simulink model "MMC_phase_centralized_HAAS_20260927"  (R2024b)
settings: Solver=FixedStepDiscrete  StartTime=t_init_sim  StopTime=sim_time  FixedStep=Ts  RelTol=1e-3
values from neighbouring files (symbols this model uses):
  a = 1    [script_MMC_phase_hackathon_NLM_centralized_HAAS_20260927.m]
  C1low1_active = 1    [script_MMC_phase_hackathon_NLM_centralized_HAAS_20260927.m]
  C2low1_active = 1    [script_MMC_phase_hackathon_NLM_centralized_HAAS_20260927.m]
  C_bus = 4400e-6    (= 0.0044)    [script_MMC_phase_hackathon_NLM_centralized_HAAS_20260927.m]
  C_M_extra = C_m-twist_high_side_C    [script_MMC_phase_hackathon_NLM_centralized_HAAS_20260927.m]
  duty_cycle = 1.0    (= 1)    [script_MMC_phase_hackathon_NLM_centralized_HAAS_20260927.m]
  f0 = 50    [script_MMC_phase_hackathon_NLM_centralized_HAAS_20260927.m]
  feeder_current_lower_rate_limit = -10    [script_MMC_phase_hackathon_NLM_centralized_HAAS_20260927.m]    (also in twist_parameters.m = -500)
  feeder_current_tab = [0.328 0.217 0.162 0.132 0.109 0.094 0.083 0.075 0.068 0.062 0.058 0.054 ... (42 elements, 14x3)]    [feeder_current.mat]
  feeder_current_upper_rate_limit = 0.386/(20e-3)    (= 19.3)    [twist_parameters.m]
  is6VExternallySupplied = true    [script_MMC_phase_hackathon_NLM_centralized_HAAS_20260927.m]
  isFeederJumperOpen = true    [script_MMC_phase_hackathon_NLM_centralized_HAAS_20260927.m]
  L_arm = 30e-3    (= 0.03)    [script_MMC_phase_hackathon_NLM_centralized_HAAS_20260927.m]
  m = 1    [script_MMC_phase_hackathon_NLM_centralized_HAAS_20260927.m]
  N = 5    [script_MMC_phase_hackathon_NLM_centralized_HAAS_20260927.m]
  power_losses = false    [script_MMC_phase_hackathon_NLM_centralized_HAAS_20260927.m]
  R = 15    [script_MMC_phase_hackathon_NLM_centralized_HAAS_20260927.m]
  R_arm = 0.2    [script_MMC_phase_hackathon_NLM_centralized_HAAS_20260927.m]
  source_V = 0    [script_MMC_phase_hackathon_NLM_centralized_HAAS_20260927.m]
  Tcom_sample = round(Tcom / Ts)    [script_MMC_phase_hackathon_NLM_centralized_HAAS_20260927.m]
  time_charge = 0.1    [script_MMC_phase_hackathon_NLM_centralized_HAAS_20260927.m]
  time_decharge = 1.5    [script_MMC_phase_hackathon_NLM_centralized_HAAS_20260927.m]
  Ts = 1e-6    (= 1e-06)    [script_MMC_phase_hackathon_NLM_centralized_HAAS_20260927.m]
  twist_data_acquisition_delay = 50e-9    (= 5e-08)    [script_MMC_phase_hackathon_NLM_centralized_HAAS_20260927.m]    (also in twist_parameters.m)
  twist_data_sampling_period = 1/twist_freq_data_sampling    (= 5e-05)    [script_MMC_phase_hackathon_NLM_centralized_HAAS_20260927.m]    (also in twist_parameters.m)
  twist_dead_time = 200e-9    (= 2e-07)    [twist_parameters.m]
  twist_freq_switching = 200e3    (= 200000)    [twist_parameters.m]
  twist_high_side_adc_R = 1/(1/2e6 + 1/2e6 + 1/(330e3+5.6e3))    (= 251272.836178)    [twist_parameters.m]
  twist_high_side_C = 33e-6*4 + 4.7e-6*12    (= 0.0001884)    [twist_parameters.m]
  twist_high_side_feeder_R = 47e3+4.7e3    (= 51700)    [twist_parameters.m]
  twist_high_side_rC = 0.1    [twist_parameters.m]
  twist_low_side_adc_R = 150e3+470    (= 150470)    [twist_parameters.m]
  twist_low_side_C_ceramic = 3*4.7e-6    (= 1.41e-05)    [twist_parameters.m]
  twist_low_side_C_electrolytic = 47e-6    (= 4.7e-05)    [twist_parameters.m]
  twist_low_side_L = 33e-6    (= 3.3e-05)    [twist_parameters.m]
  twist_low_side_rC = 700e-3    (= 0.7)    [twist_parameters.m]
  twist_low_side_rL = 20e-3    (= 0.02)    [twist_parameters.m]
  twist_R_VCC = (tau_VCC/twist_high_side_C  - twist_high_side_rC)/(1-(tau_VCC/twist_high_side_C - twist_high_side_rC)/R_parallel)    (= 1110.74997822)    [twist_parameters.m]
  VDC = 48    [script_MMC_phase_hackathon_NLM_centralized_HAAS_20260927.m]
undefined symbols (not defined in the file or in its folder): C_SM, feeder_current, gcbh, sps_rtmsupport, twist_low_side_lC
libraries: spsSeriesRLCBranchLib x135, spsTriangleGeneratorLib x60, spsMosfetLib x60, spsCurrentMeasurementLib x43, spsVoltageMeasurementLib x35, spsControlledCurrentSourceLib x30, spsDiodeLib x22, spsIdealSwitchLib x20, spsControlledVoltageSourceLib x1, spsGroundLib x1, spspowerguiLib x1
(part 1 of 22)
settings Model: Creator=ana  LastModifiedBy=ana

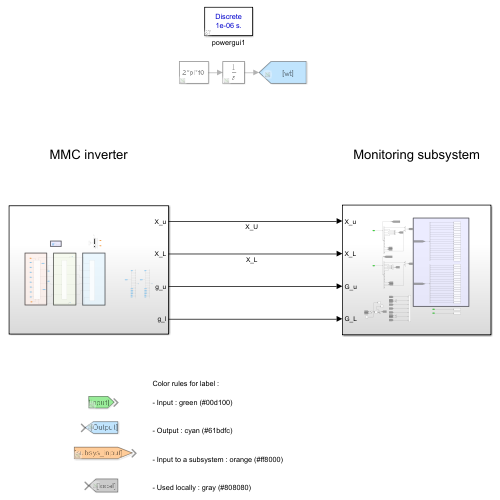
[thumbnail: Simulink's stored preview of the top-level diagram]
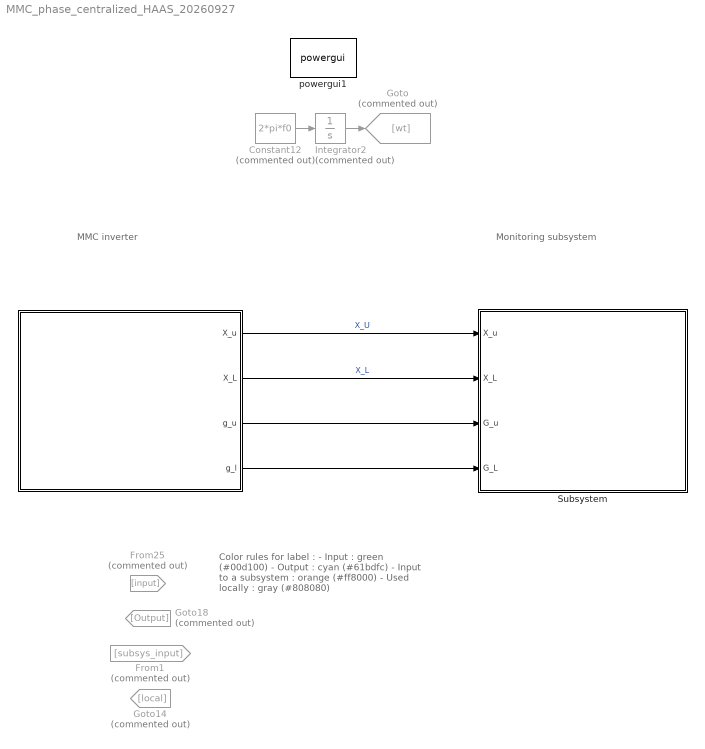
== system MMC_phase_centralized_HAAS_20260927 ==
  note: Color rules for label :
      |
      | - Input : green (#00d100)
      |
      |
      | - Output : cyan (#61bdfc)
      |
      |
      | - Input to a subsystem : orange (#ff8000)
      |
      |
      | - Used locally : gray (#808080)
  note: MMC inverter
  note: Monitoring subsystem
  " " : Subsystem
  Constant12 : Constant  Commented=on  Value=2*pi*f0
  From1 : From  Commented=on  GotoTag=subsys_input
  From25 : From  Commented=on  GotoTag=input
  Goto : Goto  Commented=on  GotoTag=wt
  Goto14 : Goto  Commented=on  GotoTag=local
  Goto18 : Goto  Commented=on  GotoTag=Output
  Integrator2 : Integrator  Commented=on
  Subsystem : Subsystem
  powergui1 : spspowerguiLib/powergui  Priority=1  SimulationMode=Discrete  SampleTime=Ts  frequency=60  Iterations=50  frequencyindice=0  Pbase=100e6  ErrMax=1e-4  UnitsV=V  UnitsW=W  buscounter=0  FunctionMessages=off  echomessages=off  EnableUseOfTLC=off  CurrentSourceSwitches=off  DisableSnubberDevices=off  DisableRonSwitches=off  DisableVfSwitches=off  DisplayEquations=off  AutomaticDiscreteSolvers=off  SolverType=Backward Euler  Interpol=off  ExternalGateDelay=off  methode=off  Ts=0  x0status=blocks  SPID=off  SwTol=0  HookPort=off  NonlinearTolerance=1e-4  nMaxIteration=100  ContinueOnMaxIteration=off  RestoreLinks=warning  ResistiveCurrentMeasurement=off  Frange=[0:2:500]  Ylog=off  Xlog=on  ShowGrid=off  save=off  variable=ZData  structure=0  ZoomFFT=off  StartTime=0.0  cycles=1  DisplayStyle=1  fundamental=60  FreqAxis=off  MaxFrequency=1000  frequencyindicesteady=1  RmsSteady=1  display=off
  wires:
  Constant12/1 -> Integrator2/1
  Integrator2/1 -> Goto/1
  " "/1(X_u) -> Subsystem/1(X_u)  "X_U"
  " "/2(X_L) -> Subsystem/2(X_L)  "X_L"
  " "/3(g_u) -> Subsystem/3(G_u)
  " "/4(g_l) -> Subsystem/4(G_L)

== system MMC_phase_centralized_HAAS_20260927/  ==
  note: Hardware
  note: Communication
  note: Power calculation
  note: Control
  Communication_subsystem : Subsystem
  Constant1 : Constant  Value=[1 1 1 1 1 1 1 1 1 1]
  Constant4 : Constant
  Constant5 : Constant  Value=[0 0 0 0 0 0 0 0 0 0]
  Demux : Demux  Outputs=10
  Demux3 : Demux  Outputs=10
  Demux4 : Demux  Outputs=10
  Mux1 : Mux  Inputs=17
  Mux{14..23} (10 alike) : Mux  Inputs=2
  Mux3 : Mux  Inputs=5
  Mux4 : Mux  Inputs=5
  Mux6 : Mux  Inputs=17
  Product1 : Product
  Sinus Modulation + Sorting Algorithm : Subsystem
      settings: PortSchema="{\"entries\":[{\"content\":{\"sides\":[{\"content\":{\"connectorIds\":[\"Out1\",\"In1\",\"In2\",\"In3\",\"In4\",\"Out2\"]},\"type\":\"ConnectorPlacement.EquallySpacedRectSide\",\"uuid\":\"ad0c70b8-bd3d-4dd9-a5c4-c9fd50c7c997\"},{\"content\":{\"side\":\"RIGHT\"},\"type\":\"ConnectorPlacement.EquallySpacedRectSide\",\"uuid\":\"9cc59a2e-07a9-40e0-b04f-27b582e27098\"},{\"content\":{\"side\":\"TOP\"},\"type\":\"ConnectorPlacement.EquallySpacedRectSide\",\"uuid\":\"c85123d6-aff8-40c6-b6df-c7fa366f0af5\"}]},\"type\":\"ConnectorPlacement.EquallySpacedConnector\",\"uuid\":\"b1891b87-83b0-4249-9289-dc35b8395afb\"}],\"packageUris\":[\"http://schema.mathworks.com/mf0/Connector/R2020b\"],\"version\":\"1.0\"}"
  Step2 : Step  Time=time_charge  SampleTime=Ts
  Subsystem : Subsystem
      settings: PortSchema="{\"entries\":[{\"content\":{\"sides\":[{\"content\":{\"connectorIds\":[\"Out7\",\"Out8\",\"Out9\",\"Out10\",\"Out11\",\"Out12\",\"Out13\",\"Out14\"]},\"type\":\"ConnectorPlacement.EquallySpacedRectSide\",\"uuid\":\"46d0b6b2-241e-4eaa-b5f4-7cb03ad6e4f0\"},{\"content\":{\"connectorIds\":[\"Out1\",\"Out2\",\"Out3\",\"Out4\",\"Out5\",\"Out6\"],\"side\":\"RIGHT\"},\"type\":\"ConnectorPlacement.EquallySpacedRectSide\",\"uuid\":\"f0391c40-5bbd-42ea-8549-0acba96c1793\"},{\"content\":{\"connectorIds\":[\"In1\",\"In2\"],\"side\":\"TOP\"},\"type\":\"ConnectorPlacement.EquallySpacedRectSide\",\"uuid\":\"1ede63b4-6869-46b3-8b67-84e7db18bcff\"},{\"content\":{\"connectorIds\":[\"In3\",\"In4\"],\"side\":\"BOTTOM\"},\"type\":\"ConnectorPlacement.EquallySpacedRectSide\",\"uuid\":\"c0e3b199-6126-45b0-9783-8fc4162e2280\"}]},\"type\":\"ConnectorPlacement.EquallySpacedConnector\",\"uuid\":\"8bedc799-aa9e-49e4-9c41-8dbcca404e51\"}],\"packageUris\":[\"http://schema.mathworks.com/mf0/Connector/R2020b\"],\"version\":\"1.0\"}"
  Switch2 : Switch  Criteria=u2 > Threshold  SaturateOnIntegerOverflow=off  InputSameDT=off
  To Workspace2 : ToWorkspace  VariableName=Pout  SaveFormat=Structure With Time  SampleTime=-1
  X_u : Outport
  X_L : Outport  Port=2
  g_u : Outport  Port=3
  g_l : Outport  Port=4
  wires:
  Mux6/1 -> X_u/1
  Sinus Modulation + Sorting Algorithm/1(gU) -> Subsystem/2(gU), g_u/1  "gU"
  Communication_subsystem/2(I_U_RX) -> Sinus Modulation + Sorting Algorithm/2(I_U)  "Iu_M1"
  Product1/1 -> To Workspace2/1  "P_sa"
  [iu] -> Product1/2
  [iu] -> Mux6/1  "Iu"
  [Vd_u] -> Mux6/12  "Vd_u"
  [N_u] -> Mux6/13  "N_u"
  [Vm_u] -> Mux6/14  "Vm_u"
  [v_a] -> Mux6/15  "V_s_a"
  [iu_M1] -> Mux6/16  "Iu_M1"
  [Vm_u] -> Product1/1
  Communication_subsystem/3(Vc_L_RX) -> Sinus Modulation + Sorting Algorithm/3(Vc_L)  "Vc_L"
  Sinus Modulation + Sorting Algorithm/2(gL) -> g_l/1, Subsystem/4(gL)  "gL"
  [il] -> Mux1/1  "iL"
  Mux1/1 -> X_L/1
  [il_M1] -> Mux1/16  "iL_M1"
  [Vd_l] -> Mux1/12  "Vd_l"
  [Vm_l] -> Mux1/14  "Vm_l"
  [N_l] -> Mux1/13  "N_l"
  [i_a] -> Mux1/15  "I_a"
  Communication_subsystem/4(I_L_RX) -> Sinus Modulation + Sorting Algorithm/4(I_L)  "IL_M1"
  Communication_subsystem/1(Vc_U_RX) -> Sinus Modulation + Sorting Algorithm/1(Vc_U)  "Vc_U"
  [Uppper_measure] -> Demux/1
  Demux/1 -> Mux6/2  "Vc_U_1"
  Demux/2 -> Mux6/3  "Vc_U_2"
  Demux/3 -> Mux6/4  "Vc_U_3"
  Demux/4 -> Mux6/5  "Vc_U_4"
  Demux/5 -> Mux6/6  "Vc_U_5"
  Demux/6 -> Mux6/7  "Vm_U_1"
  Demux/7 -> Mux6/8  "Vm_U_2"
  Demux/8 -> Mux6/9  "Vm_U_3"
  Demux/9 -> Mux6/10  "Vm_U_4"
  Demux/10 -> Mux6/11  "Vm_U_5"
  [Lower_measure] -> Demux3/1
  Demux3/1 -> Mux1/2  "Vc_L_1"
  Demux3/2 -> Mux1/3  "Vc_L_2"
  Demux3/3 -> Mux1/4  "Vc_L_3"
  Demux3/4 -> Mux1/5  "Vc_L_4"
  Demux3/5 -> Mux1/6  "Vc_L_5"
  Demux3/6 -> Mux1/7  "Vm_L_1"
  Demux3/7 -> Mux1/8  "Vm_L_2"
  Demux3/8 -> Mux1/9  "Vm_L_3"
  Demux3/9 -> Mux1/10  "Vm_L_4"
  Demux3/10 -> Mux1/11  "Vm_L_5"
  [m_u] -> Mux6/17  "m_u"
  [m_l] -> Mux1/17  "m_L"
  Subsystem/2(i_mod_M1) -> [iu_M1], Communication_subsystem/1(I_U_TX)  "IU_M1"
  Subsystem/4(i_mod_M6) -> [il_M1], Communication_subsystem/3(I_L_TX)  "IL_M6"
  Subsystem/6(Vc_L) -> Communication_subsystem/4(Vc_L_TX)
  Subsystem/3(Vc_U) -> Communication_subsystem/2(Vc_U_TX)  "Vc_U"
  Subsystem/10(i_a) -> [i_a]
  Subsystem/14(iu) -> [iu]
  Subsystem/8(Vm_u) -> [Vm_u]
  Subsystem/7(Vd_u) -> [Vd_u]
  Subsystem/12(il) -> [il]
  Subsystem/9(v_a) -> [v_a]
  Subsystem/13(Vd_l) -> [Vd_l]
  Subsystem/11(Vm_l) -> [Vm_l]
  Subsystem/5(Lower_measure) -> [Lower_measure]
  Subsystem/1(Upper_measure) -> [Uppper_measure]
  [block_U] -> Subsystem/1(block_U)
  [block_L] -> Subsystem/3(block_L)
  Demux4/9 -> Mux22/1  "block_L4"
  Mux17/1 -> Mux3/4
  Mux22/1 -> Mux4/4
  Mux14/1 -> Mux3/1
  Demux4/1 -> Mux14/1  "block_U1"
  Constant5/1 -> Switch2/1
  Demux4/3 -> Mux16/1  "block_U3"
  Mux21/1 -> Mux4/3
  Switch2/1 -> Demux4/1
  Demux4/5 -> Mux18/1  "block_U5"
  Demux4/10 -> Mux23/1  "block_L5"
  Constant1/1 -> Switch2/3
  Demux4/7 -> Mux20/1  "block_L2"
  Mux19/1 -> Mux4/1
  Mux23/1 -> Mux4/5
  Demux4/2 -> Mux15/1  "block_U2"
  Constant4/1 -> Mux23/2, Mux22/2, Mux21/2, Mux20/2, Mux19/2, Mux18/2, Mux17/2, Mux16/2, Mux15/2, Mux14/2
  Demux4/6 -> Mux19/1  "block_L1"
  Demux4/8 -> Mux21/1  "block_L3"
  Mux16/1 -> Mux3/3
  Mux15/1 -> Mux3/2
  Mux20/1 -> Mux4/2
  Mux18/1 -> Mux3/5
  Demux4/4 -> Mux17/1  "block_U4"
  Step2/1 -> Switch2/2
  Mux3/1 -> [block_U]
  Mux4/1 -> [block_L]

== system MMC_phase_centralized_HAAS_20260927/Subsystem ==
  note: To workspace
  X_u : Inport
  X_L : Inport  Port=2
  G_u : Inport  Port=3
  G_L : Inport  Port=4
  Constant : Constant  Value=2
  Demux : Demux  Outputs=2
  Demux{1..4} (4 alike) : Demux  Outputs=17
  Divide : Product  Inputs=*/
  Mux : Mux  Inputs=5
  Mux{1..3,8} (4 alike) : Mux  Inputs=2
  Mux5 : Mux  Inputs=5
  Scope : Scope
  Scope1 : Scope
  Scope3 : Scope  NumInputPorts=7
  Sum : Sum  Inputs=|++
  To Workspace1 : ToWorkspace  VariableName=vm_1  SaveFormat=Structure With Time  SampleTime=-1
  To Workspace10 : ToWorkspace  VariableName=vc_1  SaveFormat=Structure With Time  SampleTime=-1
  To Workspace11 : ToWorkspace  VariableName=va  SaveFormat=Structure With Time  SampleTime=-1
  To Workspace12 : ToWorkspace  VariableName=m_u  SaveFormat=Structure With Time  SampleTime=-1
  To Workspace13 : ToWorkspace  VariableName=i_u_M1_meas  SaveFormat=Structure With Time  SampleTime=-1
  To Workspace14 : ToWorkspace  VariableName=vm_10  SaveFormat=Structure With Time  SampleTime=-1
  To Workspace15 : ToWorkspace  VariableName=vm_2  SaveFormat=Structure With Time  SampleTime=-1
  To Workspace16 : ToWorkspace  VariableName=vm_3  SaveFormat=Structure With Time  SampleTime=-1
  To Workspace17 : ToWorkspace  VariableName=vm_4  SaveFormat=Structure With Time  SampleTime=-1
  To Workspace18 : ToWorkspace  VariableName=vm_5  SaveFormat=Structure With Time  SampleTime=-1
  To Workspace19 : ToWorkspace  VariableName=vc_10  SaveFormat=Structure With Time  SampleTime=-1
  To Workspace2 : ToWorkspace  VariableName=vc_2  SaveFormat=Structure With Time  SampleTime=-1
  To Workspace20 : ToWorkspace  VariableName=ia  SaveFormat=Structure With Time  SampleTime=-1
  To Workspace21 : ToWorkspace  VariableName=m_l  SaveFormat=Structure With Time  SampleTime=-1
  To Workspace22 : ToWorkspace  VariableName=i_l_M1_meas  SaveFormat=Structure With Time  SampleTime=-1
  To Workspace23 : ToWorkspace  VariableName=vm_6  SaveFormat=Structure With Time  SampleTime=-1
  To Workspace24 : ToWorkspace  VariableName=vm_7  SaveFormat=Structure With Time  SampleTime=-1
  To Workspace25 : ToWorkspace  VariableName=vm_8  SaveFormat=Structure With Time  SampleTime=-1
  To Workspace26 : ToWorkspace  VariableName=vm_9  SaveFormat=Structure With Time  SampleTime=-1
  To Workspace27 : ToWorkspace  VariableName=vc_6  SaveFormat=Structure With Time  SampleTime=-1
  To Workspace28 : ToWorkspace  VariableName=vc_7  SaveFormat=Structure With Time  SampleTime=-1
  To Workspace29 : ToWorkspace  VariableName=vc_8  SaveFormat=Structure With Time  SampleTime=-1
  To Workspace3 : ToWorkspace  VariableName=vc_3  SaveFormat=Structure With Time  SampleTime=-1
  To Workspace30 : ToWorkspace  VariableName=vc_9  SaveFormat=Structure With Time  SampleTime=-1
  To Workspace31 : ToWorkspace  VariableName=vd_l  SaveFormat=Structure With Time  SampleTime=-1
  To Workspace32 : ToWorkspace  VariableName=N_l  SaveFormat=Structure With Time  SampleTime=-1
  To Workspace33 : ToWorkspace  VariableName=i_l  SaveFormat=Structure With Time  SampleTime=-1
  To Workspace34 : ToWorkspace  VariableName=vm_l  SaveFormat=Structure With Time  SampleTime=-1
  To Workspace35 : ToWorkspace  VariableName=g_u  SaveFormat=Structure With Time  SampleTime=-1
  To Workspace36 : ToWorkspace  VariableName=g_L  SaveFormat=Structure With Time  SampleTime=-1
  To Workspace4 : ToWorkspace  VariableName=vc_4  SaveFormat=Structure With Time  SampleTime=-1
  To Workspace5 : ToWorkspace  VariableName=vc_5  SaveFormat=Structure With Time  SampleTime=-1
  To Workspace6 : ToWorkspace  VariableName=vd_u  SaveFormat=Structure With Time  SampleTime=-1
  To Workspace7 : ToWorkspace  VariableName=N_u  SaveFormat=Structure With Time  SampleTime=-1
  To Workspace8 : ToWorkspace  VariableName=i_u  SaveFormat=Structure With Time  SampleTime=-1
  To Workspace9 : ToWorkspace  VariableName=vm_u  SaveFormat=Structure With Time  SampleTime=-1
  wires:
  Demux4/15 -> To Workspace20/1  "i_a"
  Demux1/4 -> To Workspace3/1  "Vc_3"
  Demux4/17 -> To Workspace21/1  "m_l"
  X_L/1 -> Demux3/1, [l_SW]
  Demux2/14 -> [v_m_u]  "Vm_u"
  Demux1/2 -> To Workspace10/1  "Vc_1"
  Demux1/14 -> To Workspace9/1  "Vm_u"
  Mux2/1 -> Scope3/2  "V_m_U/L"
  Demux4/3 -> To Workspace28/1  "Vc_2"
  Demux1/7 -> To Workspace1/1  "Vm_1"
  Demux4/1 -> To Workspace33/1  "i_l"
  Demux2/1 -> Mux3/1  "i_u"
  Demux2/4 -> Mux/3  "V_uc_3"
  [v_m_u] -> Mux2/1
  [i_a] -> Scope3/7  "I_a"
  X_u/1 -> Demux2/1, [u_SW]
  Demux2/15 -> [v_a]  "V_a"
  Demux3/6 -> Mux5/5  "Vc_l_5"
  Demux2/16 -> Mux3/2  "iu_M1_meas"
  [i_l] -> Sum/2
  Demux3/1 -> Mux8/1  "i_l"
  Demux4/7 -> To Workspace23/1  "Vm_1"
  Demux1/11 -> To Workspace18/1  "Vm_5"
  Demux3/16 -> Mux8/2  "il_M1_meas"
  Demux1/13 -> To Workspace7/1  "N_u"
  Demux4/9 -> To Workspace25/1  "Vm_3"
  Demux2/3 -> Mux/2  "Vc_u_2"
  [i_u] -> Mux1/1
  Demux4/11 -> To Workspace14/1  "Vm_5"
  Mux5/1 -> [v_c_l]
  Demux4/8 -> To Workspace24/1  "Vm_2"
  [l_SW] -> Demux4/1  "L_SW"
  Demux1/5 -> To Workspace4/1  "Vc_4"
  Mux8/1 -> [i_l]
  Mux3/1 -> [i_u]  "I_u"
  Demux3/3 -> Mux5/2  "Vc_l_2"
  Constant/1 -> Divide/2
  Demux3/5 -> Mux5/4  "Vc_l_4"
  Demux4/4 -> To Workspace29/1  "Vc_3"
  Sum/1 -> Scope1/1, Divide/1  "I_u + I_L"
  Demux3/15 -> [i_a]  "i_a"
  Divide/1 -> Scope/1, Demux/1  "(I_U + I_L)/2"
  Demux1/3 -> To Workspace2/1  "Vc_2"
  Demux3/2 -> Mux5/1  "Vc_l_1"
  Demux1/16 -> To Workspace13/1  "iu_M1_meas"
  Demux2/5 -> Mux/4  "Vc_u_4"
  [v_a] -> Scope3/3  "V_a"
  Demux4/16 -> To Workspace22/1  "il_M1_meas"
  Demux1/10 -> To Workspace17/1  "Vm_4"
  [i_l] -> Mux1/2
  [u_SW] -> Demux1/1  "u_SW"
  Demux1/17 -> To Workspace12/1  "m_u"
  Demux1/15 -> To Workspace11/1  "Va"
  Demux1/12 -> To Workspace6/1  "Vd_u"
  Demux2/2 -> Mux/1  "Vc_u_1"
  Demux4/13 -> To Workspace32/1  "N_l"
  Demux1/9 -> To Workspace16/1  "Vm_3"
  Demux4/6 -> To Workspace19/1  "Vc_5"
  Demux4/2 -> To Workspace27/1  "Vc_1"
  Demux4/14 -> To Workspace34/1  "Vm_l"
  Demux/1 -> [i_Sigma_a]
  [v_c_l] -> Scope3/5  "V_c_L"
  Demux2/6 -> Mux/5  "Vc_u_5"
  Demux1/8 -> To Workspace15/1  "Vm_2"
  [v_c_u] -> Scope3/1  "V_c_u"
  Demux1/6 -> To Workspace5/1  "Vc_5"
  Demux1/1 -> To Workspace8/1  "i_u"
  [v_m_l] -> Mux2/2
  [i_u] -> Sum/1
  [i_Sigma_a] -> Scope3/4  "i_Sigma"
  Demux4/12 -> To Workspace31/1  "Vd_l"
  Demux3/14 -> [v_m_l]  "Vm_l"
  Mux1/1 -> Scope3/6  "I_U/L"
  Demux3/4 -> Mux5/3  "Vc_l_3"
  Mux/1 -> [v_c_u]  "V_c_u"
  Demux4/10 -> To Workspace26/1  "Vm_4"
  Demux4/5 -> To Workspace30/1  "Vc_4"
  G_u/1 -> To Workspace35/1
  G_L/1 -> To Workspace36/1

== system MMC_phase_centralized_HAAS_20260927/ /Communication_subsystem ==
  I_U_TX : Inport
  Vc_U_TX : Inport  Port=2
  I_L_TX : Inport  Port=3
  Vc_L_TX : Inport  Port=4
  Communication architecture : Subsystem
      settings: PortSchema="{\"entries\":[{\"content\":{\"sides\":[{\"content\":{\"connectorIds\":[\"In1\",\"Out2\",\"In2\",\"Out3\",\"In3\",\"Out4\",\"In4\",\"Out5\",\"In5\",\"Out6\",\"In6\",\"Out7\",\"In7\",\"Out8\",\"In8\",\"Out9\",\"In9\",\"Out10\",\"In10\",\"Out11\"]},\"type\":\"ConnectorPlacement.EquallySpacedRectSide\",\"uuid\":\"574f1c32-5c90-4713-aad2-348eca17c1e3\"},{\"content\":{\"connectorIds\":[\"Out1\"],\"side\":\"RIGHT\"},\"type\":\"ConnectorPlacement.EquallySpacedRectSide\",\"uuid\":\"f8c779b5-ecb7-4a42-bc9c-e4bb2f97a0b3\"},{\"content\":{\"side\":\"TOP\"},\"type\":\"ConnectorPlacement.EquallySpacedRectSide\",\"uuid\":\"aac8d141-a504-4135-a079-04baa73dba14\"}]},\"type\":\"ConnectorPlacement.EquallySpacedConnector\",\"uuid\":\"cbc34fff-d47b-42f9-bfde-18f06952df39\"}],\"packageUris\":[\"http://schema.mathworks.com/mf0/Connector/R2020b\"],\"version\":\"1.0\"}"
  Demux2 : Demux  Outputs=12
  Lower_arm : Subsystem
      settings: PortSchema="{\"entries\":[{\"content\":{\"sides\":[{\"content\":{\"connectorIds\":[\"In1\",\"In2\"]},\"type\":\"ConnectorPlacement.EquallySpacedRectSide\",\"uuid\":\"bca47161-c2bf-4caa-811b-3e74c86277e3\"},{\"content\":{\"connectorIds\":[\"Out1\",\"In3\",\"Out2\",\"In4\",\"Out3\",\"In5\",\"Out4\",\"In6\",\"Out5\",\"In7\"],\"side\":\"RIGHT\"},\"type\":\"ConnectorPlacement.EquallySpacedRectSide\",\"uuid\":\"b2e32fb7-723a-4edb-b512-e2e9b6c6de33\"},{\"content\":{\"side\":\"TOP\"},\"type\":\"ConnectorPlacement.EquallySpacedRectSide\",\"uuid\":\"c04e7617-ef7b-4140-bc2d-a2cc51392c69\"}]},\"type\":\"ConnectorPlacement.EquallySpacedConnector\",\"uuid\":\"316a164c-4e23-40e3-8762-9cd74b77f738\"}],\"packageUris\":[\"http://schema.mathworks.com/mf0/Connector/R2020b\"],\"version\":\"1.0\"}"
  Mux : Mux  Inputs=2
  Mux1 : Mux  Inputs=2
  Scope : Scope
  Sync : DiscretePulseGenerator  Period=round((200e-6)/Ts)  PulseWidth=round(20e-6/Ts)  SampleTime=Ts
  Upper_arm : Subsystem
      settings: PortSchema="{\"entries\":[{\"content\":{\"sides\":[{\"content\":{\"connectorIds\":[\"In1\",\"In2\"]},\"type\":\"ConnectorPlacement.EquallySpacedRectSide\",\"uuid\":\"e2448297-5920-4ed4-b9a5-463387ed0389\"},{\"content\":{\"connectorIds\":[\"Out1\",\"In3\",\"Out2\",\"In4\",\"Out3\",\"In5\",\"Out4\",\"In6\",\"Out5\",\"In7\"],\"side\":\"RIGHT\"},\"type\":\"ConnectorPlacement.EquallySpacedRectSide\",\"uuid\":\"29ac6558-0bf6-4432-86a8-2cc792ef1820\"},{\"content\":{\"connectorIds\":[\"Out6\"],\"side\":\"TOP\"},\"type\":\"ConnectorPlacement.EquallySpacedRectSide\",\"uuid\":\"fe3a666d-35d9-4a5d-8998-edcd1cd24e1f\"}]},\"type\":\"ConnectorPlacement.EquallySpacedConnector\",\"uuid\":\"a9564cd0-ea30-4b39-994d-f524846fcfc7\"}],\"packageUris\":[\"http://schema.mathworks.com/mf0/Connector/R2020b\"],\"version\":\"1.0\"}"
  Vector Concatenate : Concatenate  NumInputs=5
  Vector Concatenate1 : Concatenate  NumInputs=5
  Vc_U_RX : Outport
  I_U_RX : Outport  Port=2
  Vc_L_RX : Outport  Port=3
  I_L_RX : Outport  Port=4
  wires:
  Vc_U_TX/1 -> Mux/1
  Mux/1 -> Upper_arm/1(upper_arm_info)
  Vc_L_TX/1 -> Mux1/1
  I_L_TX/1 -> Mux1/2
  Mux1/1 -> Lower_arm/2(lower_arm_info)
  Upper_arm/1(M1_TX_signal) -> Communication architecture/1(M1_TX_Signal)
  Upper_arm/2(M2_TX_signal) -> Communication architecture/2(M2_TX_Signal)
  Upper_arm/3(M3_TX_signal) -> Communication architecture/3(M3_TX_Signal)
  Upper_arm/4(M4_TX_signal) -> Communication architecture/4(M4_TX_Signal)
  Upper_arm/5(M5_TX_signal) -> Communication architecture/5(M5_TX_Signal)
  Lower_arm/1(M6_TX_signal) -> Communication architecture/6(M6_TX_Signal)
  Lower_arm/2(M7_TX_signal) -> Communication architecture/7(M7_TX_Signal)
  Lower_arm/3(M8_TX_signal) -> Communication architecture/8(M8_TX_Signal)
  Lower_arm/4(M9_TX_signal) -> Communication architecture/9(M9_TX_Signal)
  Lower_arm/5(M10_TX_signal) -> Communication architecture/10(M10_TX_Signal)
  I_U_TX/1 -> Mux/2
  Sync/1 -> Lower_arm/1(sync), Upper_arm/2(sync)
  Upper_arm/6(RX_Variables) -> [RX_variable]
  [RX_variable] -> Demux2/1
  Demux2/1 -> Scope/1, Vector Concatenate/1  "Vc_u_1"
  Demux2/2 -> Vector Concatenate/2  "Vc_u_2"
  Demux2/3 -> Vector Concatenate/3  "Vc_u_3"
  Demux2/4 -> Vector Concatenate/4  "Vc_u_4"
  Demux2/5 -> Vector Concatenate/5  "Vc_u_5"
  Vector Concatenate/1 -> Vc_U_RX/1
  Demux2/6 -> I_U_RX/1
  Demux2/11 -> Vector Concatenate1/5  "Vc_l_5"
  Demux2/9 -> Vector Concatenate1/3  "Vc_l_3"
  Demux2/8 -> Vector Concatenate1/2  "Vc_l_2"
  Demux2/10 -> Vector Concatenate1/4  "Vc_l_4"
  Demux2/7 -> Vector Concatenate1/1  "Vc_l_1"
  Vector Concatenate1/1 -> Vc_L_RX/1
  Demux2/12 -> I_L_RX/1
  Communication architecture/2(M1_RX_Signal) -> Upper_arm/3(M1_RX_signal)
  Communication architecture/3(M2_RX_Signal) -> Upper_arm/4(M2_RX_signal)
  Communication architecture/4(M3_RX_Signal) -> Upper_arm/5(M3_RX_signal)
  Communication architecture/5(M4_RX_Signal) -> Upper_arm/6(M4_RX_signal)
  Communication architecture/6(M5_RX_Signal) -> Upper_arm/7(M5_RX_signal)
  Communication architecture/7(M6_RX_Signal) -> Lower_arm/3(M6_RX_signal)
  Communication architecture/8(M7_RX_Signal) -> Lower_arm/4(M7_RX_signal)
  Communication architecture/9(M8_RX_Signal) -> Lower_arm/5(M8_RX_signal)
  Communication architecture/10(M9_RX_Signal) -> Lower_arm/6(M9_RX_signal)
  Communication architecture/11(M10_RX_Signal) -> Lower_arm/7(M10_RX_signal)

== system MMC_phase_centralized_HAAS_20260927/ /Sinus Modulation + Sorting Algorithm ==
  note: Sorting and CVB algorithm - Upper and Lower stacks
  note: Gate assignement - Modules MCUs
  Vc_U : Inport
  I_U : Inport  Port=2
  Vc_L : Inport  Port=3
  I_L : Inport  Port=4
  Constant10 : Constant
  Constant11 : Constant  Value=2
  Constant12 : Constant  Value=3
  Constant13 : Constant  Value=4
  Constant14 : Constant  Value=5
  Constant5 : Constant
  Constant6 : Constant  Value=2
  Constant7 : Constant  Value=3
  Constant8 : Constant  Value=4
  Constant9 : Constant  Value=5
  M1 MCU : Subsystem
  M2 MCU : Subsystem
  M3 MCU : Subsystem
  M4 MCU : Subsystem
  M5 MCU : Subsystem
  M5 MCU1 : Subsystem
  M5 MCU2 : Subsystem
  M5 MCU3 : Subsystem
  M5 MCU4 : Subsystem
  M5 MCU5 : Subsystem
  Mux : Mux  Inputs=5
  Mux1 : Mux  Inputs=5
  Supervisor MCU : Subsystem
  gU : Outport
  gL : Outport  Port=2
  tag scope: g_l_supervisor=global, g_u_supervisor=global
  wires:
  M1 MCU/1(g_unitaire_stack) -> Mux/1
  M2 MCU/1(g_unitaire_stack) -> Mux/2
  M3 MCU/1(g_unitaire_stack) -> Mux/3
  M4 MCU/1(g_unitaire_stack) -> Mux/4
  M5 MCU/1(g_unitaire_stack) -> Mux/5
  Constant5/1 -> M1 MCU/2(M_number)
  Constant6/1 -> M2 MCU/2(M_number)
  Constant7/1 -> M3 MCU/2(M_number)
  Constant8/1 -> M4 MCU/2(M_number)
  Constant9/1 -> M5 MCU/2(M_number)
  M5 MCU3/1(g_unitaire_stack) -> Mux1/3
  M5 MCU4/1(g_unitaire_stack) -> Mux1/4
  M5 MCU5/1(g_unitaire_stack) -> Mux1/5
  Constant10/1 -> M5 MCU1/2(M_number)
  Constant11/1 -> M5 MCU2/2(M_number)
  Constant12/1 -> M5 MCU3/2(M_number)
  Constant13/1 -> M5 MCU4/2(M_number)
  Constant14/1 -> M5 MCU5/2(M_number)
  I_U/1 -> Supervisor MCU/2(I_U)
  Vc_U/1 -> Supervisor MCU/1(Vc_U)
  Vc_L/1 -> Supervisor MCU/3(Vc_L)
  I_L/1 -> Supervisor MCU/4(I_L)
  M5 MCU1/1(g_unitaire_stack) -> Mux1/1
  M5 MCU2/1(g_unitaire_stack) -> Mux1/2
  Supervisor MCU/1(gU) -> [g_u_supervisor]
  Supervisor MCU/2(gL) -> [g_l_supervisor]
  [g_u_supervisor] -> M5 MCU/1(g_u), M4 MCU/1(g_u), M3 MCU/1(g_u), M2 MCU/1(g_u), M1 MCU/1(g_u)
  [g_l_supervisor] -> M5 MCU5/1(g_u), M5 MCU4/1(g_u), M5 MCU3/1(g_u), M5 MCU2/1(g_u), M5 MCU1/1(g_u)
  Mux1/1 -> gL/1
  Mux/1 -> gU/1

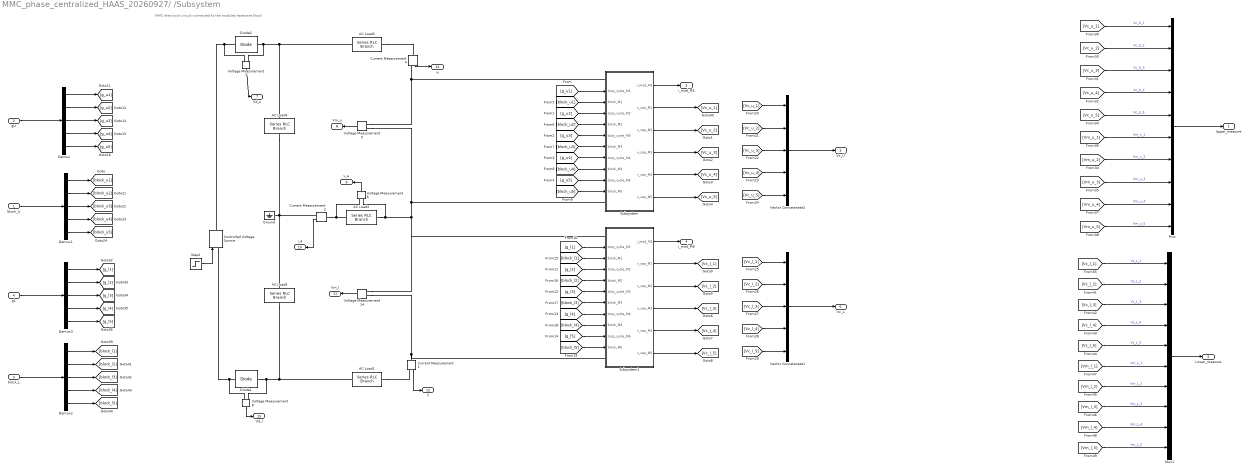
== system MMC_phase_centralized_HAAS_20260927/ /Subsystem ==
  note: MMC electrical circuit connected to the modules hardware block
  block_U : Inport
  gU : Inport  Port=2
  block_L : Inport  Port=3
  gL : Inport  Port=4
  AC Load1 : spsSeriesRLCBranchLib/Series RLC Branch  LConnTagsString=__new0  RConnTagsString=__new0  BranchType=RL  Resistance=R_arm  Inductance=L_arm  SetiL0=off  InitialCurrent=0  Capacitance=C_SM  Setx0=off  InitialVoltage=0  Measurements=None
  AC Load2 : spsSeriesRLCBranchLib/Series RLC Branch  LConnTagsString=__new0  RConnTagsString=__new0  BranchType=RL  Resistance=R_arm  Inductance=L_arm  SetiL0=off  InitialCurrent=0  Capacitance=C_SM  Setx0=off  InitialVoltage=0  Measurements=None
  AC Load3 : spsSeriesRLCBranchLib/Series RLC Branch  LConnTagsString=__new0  RConnTagsString=__new0  BranchType=R  Resistance=R  Inductance=L_arm  SetiL0=off  InitialCurrent=0  Capacitance=C_SM  Setx0=off  InitialVoltage=0  Measurements=None
  AC Load4 : spsSeriesRLCBranchLib/Series RLC Branch  LConnTagsString=__new0  RConnTagsString=__new0  BranchType=C  Resistance=R  Inductance=L_arm  SetiL0=off  InitialCurrent=0  Capacitance=C_bus  Setx0=off  InitialVoltage=0  Measurements=None
  AC Load5 : spsSeriesRLCBranchLib/Series RLC Branch  LConnTagsString=__new0  RConnTagsString=__new0  BranchType=C  Resistance=R  Inductance=L_arm  SetiL0=off  InitialCurrent=0  Capacitance=C_bus  Setx0=off  InitialVoltage=0  Measurements=None
  Controlled Voltage Source : spsControlledVoltageSourceLib/Controlled Voltage Source  Initialize=on  Source_Type=DC  Amplitude=0  Phase=0  Frequency=0  Measurements=None
  Current Measurement1 : spsCurrentMeasurementLib/Current Measurement  PhasorSimulation=off  OutputType=Complex  PSBequivalent=0
  Current Measurement2 : spsCurrentMeasurementLib/Current Measurement  PhasorSimulation=off  OutputType=Complex  PSBequivalent=0
  Current Measurement4 : spsCurrentMeasurementLib/Current Measurement  PhasorSimulation=off  OutputType=Complex  PSBequivalent=0
  Demux{,1..3} (4 alike) : Demux  Outputs=5
  Diode1 : spsDiodeLib/Diode  Ron=0.001  Lon=0  Vf=0.8  IC=0  UseSnubber=0  Rs=1e5  Cs=inf  Measurements=off
  Diode2 : spsDiodeLib/Diode  Ron=0.001  Lon=0  Vf=0.8  IC=0  UseSnubber=0  Rs=1e5  Cs=inf  Measurements=off
  Ground : spsGroundLib/Ground  LConnTagsString=a
  Mux : Mux  Inputs=10
  Mux1 : Mux  Inputs=10
  Step2 : Step  Time=time_decharge  Before=VDC  After=0  SampleTime=0
  Subsystem : Subsystem
      settings: PortSchema="{\"entries\":[{\"content\":{\"sides\":[{\"content\":{\"connectorIds\":[\"LConn1\",\"In1\",\"In2\",\"In3\",\"In4\",\"In5\",\"In6\",\"In7\",\"In8\",\"In9\",\"In10\",\"LConn2\"]},\"type\":\"ConnectorPlacement.EquallySpacedRectSide\",\"uuid\":\"af96ca56-9fdb-47ea-8e31-50f481daafc4\"},{\"content\":{\"connectorIds\":[\"Out1\",\"Out2\",\"Out3\",\"Out4\",\"Out5\",\"Out6\"],\"side\":\"RIGHT\"},\"type\":\"ConnectorPlacement.EquallySpacedRectSide\",\"uuid\":\"66f6256f-049a-4c8a-aad5-8d93b148b037\"},{\"content\":{\"side\":\"TOP\"},\"type\":\"ConnectorPlacement.EquallySpacedRectSide\",\"uuid\":\"596eb3e1-7761-4783-802e-d9df31b3a9c1\"}]},\"type\":\"ConnectorPlacement.EquallySpacedConnector\",\"uuid\":\"34c6ade5-a2f4-48d8-9a9b-6856a5a88d76\"}],\"packageUris\":[\"http://schema.mathworks.com/mf0/Connector/R2020b\"],\"version\":\"1.0\"}"
  Subsystem1 : Subsystem
      settings: PortSchema="{\"entries\":[{\"content\":{\"sides\":[{\"content\":{\"connectorIds\":[\"LConn1\",\"In1\",\"In2\",\"In3\",\"In4\",\"In5\",\"In6\",\"In7\",\"In8\",\"In9\",\"In10\",\"LConn2\"]},\"type\":\"ConnectorPlacement.EquallySpacedRectSide\",\"uuid\":\"af96ca56-9fdb-47ea-8e31-50f481daafc4\"},{\"content\":{\"connectorIds\":[\"Out1\",\"Out2\",\"Out3\",\"Out4\",\"Out5\",\"Out6\"],\"side\":\"RIGHT\"},\"type\":\"ConnectorPlacement.EquallySpacedRectSide\",\"uuid\":\"66f6256f-049a-4c8a-aad5-8d93b148b037\"},{\"content\":{\"side\":\"TOP\"},\"type\":\"ConnectorPlacement.EquallySpacedRectSide\",\"uuid\":\"596eb3e1-7761-4783-802e-d9df31b3a9c1\"}]},\"type\":\"ConnectorPlacement.EquallySpacedConnector\",\"uuid\":\"34c6ade5-a2f4-48d8-9a9b-6856a5a88d76\"}],\"packageUris\":[\"http://schema.mathworks.com/mf0/Connector/R2020b\"],\"version\":\"1.0\"}"
  Vector Concatenate1 : Concatenate  NumInputs=5
  Vector Concatenate2 : Concatenate  NumInputs=5
  Voltage Measurement{5..8,14} (5 alike) : spsVoltageMeasurementLib/Voltage Measurement  PhasorSimulation=off  OutputType=Complex  PSBequivalent=0
  Upper_measure : Outport
  i_mod_M1 : Outport  Port=2
  Vc_U : Outport  Port=3
  i_mod_M6 : Outport  Port=4
  Lower_measure : Outport  Port=5
  Vc_L : Outport  Port=6
  Vd_u : Outport  Port=7
  Vm_u : Outport  Port=8
  v_a : Outport  Port=9
  i_a : Outport  Port=10
  Vm_l : Outport  Port=11
  il : Outport  Port=12
  Vd_l : Outport  Port=13
  iu : Outport  Port=14
  wires:
  Voltage Measurement7/1 -> Vd_u/1
  Current Measurement2/1 -> i_a/1
  Step2/1 -> Controlled Voltage Source/1
  Voltage Measurement5/1 -> Vm_u/1
  Voltage Measurement6/1 -> v_a/1
  Voltage Measurement14/1 -> Vm_l/1
  [g_u1] -> Subsystem/1(duty_cycle_M1)
  [block_u1] -> Subsystem/2(block_M1)
  [g_u2] -> Subsystem/3(duty_cycle_M2)
  [block_u2] -> Subsystem/4(block_M2)
  [g_u3] -> Subsystem/5(duty_cycle_M3)
  [block_u3] -> Subsystem/6(block_M3)
  [g_u4] -> Subsystem/7(duty_cycle_M4)
  [block_u4] -> Subsystem/8(block_M4)
  [g_u5] -> Subsystem/9(duty_cycle_M5)
  [block_u5] -> Subsystem/10(block_M5)
  Subsystem/1(i_mod_M1) -> i_mod_M1/1
  Subsystem/6(v_cap_M5) -> [Vc_u_5]
  Subsystem/5(v_cap_M4) -> [Vc_u_4]
  Subsystem/2(v_cap_M1) -> [Vc_u_1]
  Subsystem/3(v_cap_M2) -> [Vc_u_2]
  Subsystem/4(v_cap_M3) -> [Vc_u_3]
  [block_l4] -> Subsystem1/8(block_M4)
  [g_l4] -> Subsystem1/7(duty_cycle_M4)
  [block_l5] -> Subsystem1/10(block_M5)
  [g_l5] -> Subsystem1/9(duty_cycle_M5)
  [g_l1] -> Subsystem1/1(duty_cycle_M1)
  [g_l2] -> Subsystem1/3(duty_cycle_M2)
  [block_l2] -> Subsystem1/4(block_M2)
  [g_l3] -> Subsystem1/5(duty_cycle_M3)
  [block_l1] -> Subsystem1/2(block_M1)
  [block_l3] -> Subsystem1/6(block_M3)
  Subsystem1/1(i_mod_M1) -> i_mod_M6/1
  Subsystem1/2(v_cap_M1) -> [Vc_l_1]
  Subsystem1/3(v_cap_M2) -> [Vc_l_2]
  Subsystem1/4(v_cap_M3) -> [Vc_l_3]
  Subsystem1/5(v_cap_M4) -> [Vc_l_4]
  Subsystem1/6(v_cap_M5) -> [Vc_l_5]
  Current Measurement4/1 -> iu/1
  Voltage Measurement8/1 -> Vd_l/1
  Current Measurement1/1 -> il/1
  Vector Concatenate2/1 -> Vc_U/1
  Demux/2 -> [g_u2]
  Demux/5 -> [g_u5]
  Demux1/5 -> [block_u5]
  Demux/4 -> [g_u4]
  Demux/3 -> [g_u3]
  Demux1/1 -> [block_u1]
  gU/1 -> Demux/1
  block_U/1 -> Demux1/1
  Demux1/2 -> [block_u2]
  Demux/1 -> [g_u1]
  Demux1/4 -> [block_u4]
  Demux1/3 -> [block_u3]
  Demux3/3 -> [g_l3]
  Demux3/4 -> [g_l4]
  Demux2/3 -> [block_l3]
  Demux2/1 -> [block_l1]
  Demux3/1 -> [g_l1]
  gL/1 -> Demux3/1
  Demux2/2 -> [block_l2]
  Demux2/4 -> [block_l4]
  Demux2/5 -> [block_l5]
  Demux3/5 -> [g_l5]
  block_L/1 -> Demux2/1
  Demux3/2 -> [g_l2]
  [Vc_u_1] -> Vector Concatenate2/1
  [Vc_u_2] -> Vector Concatenate2/2
  [Vc_u_3] -> Vector Concatenate2/3
  [Vc_u_4] -> Vector Concatenate2/4
  [Vc_u_5] -> Vector Concatenate2/5
  [Vc_l_5] -> Vector Concatenate1/5
  [Vc_l_1] -> Vector Concatenate1/1
  [Vc_l_4] -> Vector Concatenate1/4
  Vector Concatenate1/1 -> Vc_L/1
  [Vc_l_3] -> Vector Concatenate1/3
  [Vc_l_2] -> Vector Concatenate1/2
  [Vc_u_1] -> Mux/1  "Vc_U_1"
  [Vm_u_5] -> Mux/10  "Vm_u_5"
  [Vm_u_4] -> Mux/9  "Vm_u_4"
  [Vc_u_3] -> Mux/3  "Vc_U_3"
  [Vm_u_3] -> Mux/8  "Vm_u_3"
  [Vc_u_2] -> Mux/2  "Vc_U_2"
  [Vm_u_2] -> Mux/7  "Vm_u_2"
  [Vm_u_1] -> Mux/6  "Vm_u_1"
  [Vc_u_4] -> Mux/4  "Vc_U_4"
  [Vc_u_5] -> Mux/5  "Vc_U_5"
  [Vc_l_2] -> Mux1/2  "Vc_L_2"
  [Vm_l_2] -> Mux1/7  "Vm_L_2"
  [Vc_l_1] -> Mux1/1  "Vc_L_1"
  [Vm_l_4] -> Mux1/9  "Vm_L_4"
  [Vm_l_5] -> Mux1/10  "Vm_L_5"
  [Vm_l_1] -> Mux1/6  "Vm_L_1"
  [Vm_l_3] -> Mux1/8  "Vm_L_3"
  [Vc_l_3] -> Mux1/3  "Vc_L_3"
  [Vc_l_5] -> Mux1/5  "Vc_L_5"
  [Vc_l_4] -> Mux1/4  "Vc_L_4"
  Mux1/1 -> Lower_measure/1
  Mux/1 -> Upper_measure/1
  connections:
  Controlled Voltage Source/LConn1 -- Voltage Measurement8/LConn2 -- Diode1/RConn1
  AC Load2/LConn1 -- AC Load4/LConn1 -- Diode2/RConn1 -- Voltage Measurement7/LConn2
  Current Measurement4/RConn1 -- Voltage Measurement5/LConn1 -- Subsystem/LConn1
  Voltage Measurement14/LConn2 -- Subsystem1/LConn2 -- Current Measurement1/LConn1
  AC Load2/RConn1 -- Current Measurement4/LConn1
  Voltage Measurement6/LConn1 -- Subsystem1/LConn1 -- Voltage Measurement14/LConn1 -- Voltage Measurement5/LConn2 -- Subsystem/LConn2 -- AC Load3/RConn1
  Ground/LConn1 -- AC Load5/LConn1 -- AC Load4/RConn1 -- Current Measurement2/RConn1
  AC Load1/RConn1 -- Current Measurement1/RConn1
  Voltage Measurement7/LConn1 -- Controlled Voltage Source/RConn1 -- Diode2/LConn1
  AC Load1/LConn1 -- Diode1/LConn1 -- Voltage Measurement8/LConn1 -- AC Load5/RConn1
  Current Measurement2/LConn1 -- Voltage Measurement6/LConn2 -- AC Load3/LConn1

== system MMC_phase_centralized_HAAS_20260927/ /Communication_subsystem/Communication architecture ==
  M1_TX_Signal : Inport
  M2_TX_Signal : Inport  Port=2
  M3_TX_Signal : Inport  Port=3
  M4_TX_Signal : Inport  Port=4
  M5_TX_Signal : Inport  Port=5
  M6_TX_Signal : Inport  Port=6
  M7_TX_Signal : Inport  Port=7
  M8_TX_Signal : Inport  Port=8
  M9_TX_Signal : Inport  Port=9
  M10_TX_Signal : Inport  Port=10
  MATLAB Function : MATLAB Function  Commented=on  TreatAsAtomicUnit=on
  RX_Signal : Outport
  M1_RX_Signal : Outport  Port=2
  M2_RX_Signal : Outport  Port=3
  M3_RX_Signal : Outport  Port=4
  M4_RX_Signal : Outport  Port=5
  M5_RX_Signal : Outport  Port=6
  M6_RX_Signal : Outport  Port=7
  M7_RX_Signal : Outport  Port=8
  M8_RX_Signal : Outport  Port=9
  M9_RX_Signal : Outport  Port=10
  M10_RX_Signal : Outport  Port=11
  wires:
  MATLAB Function/1(bus_signal) -> RX_Signal/1
  M4_TX_Signal/1 -> M5_RX_Signal/1
  M5_TX_Signal/1 -> M6_RX_Signal/1
  M6_TX_Signal/1 -> M7_RX_Signal/1
  M7_TX_Signal/1 -> M8_RX_Signal/1
  M8_TX_Signal/1 -> M9_RX_Signal/1
  M9_TX_Signal/1 -> M10_RX_Signal/1
  M10_TX_Signal/1 -> M1_RX_Signal/1
  M1_TX_Signal/1 -> M2_RX_Signal/1
  M2_TX_Signal/1 -> M3_RX_Signal/1
  M3_TX_Signal/1 -> M4_RX_Signal/1

== system MMC_phase_centralized_HAAS_20260927/ /Communication_subsystem/Lower_arm ==
  sync : Inport
  lower_arm_info : Inport  Port=2
  M6_RX_signal : Inport  Port=3
  M7_RX_signal : Inport  Port=4
  M8_RX_signal : Inport  Port=5
  M9_RX_signal : Inport  Port=6
  M10_RX_signal : Inport  Port=7
  M1_Comm : Subsystem
      settings: PortSchema="{\"entries\":[{\"content\":{\"sides\":[{\"content\":{\"connectorIds\":[\"In1\",\"Out2\"]},\"type\":\"ConnectorPlacement.EquallySpacedRectSide\",\"uuid\":\"47077a1e-eba1-4129-8203-93262b2de465\"},{\"content\":{\"connectorIds\":[\"Out1\",\"In3\"],\"side\":\"RIGHT\"},\"type\":\"ConnectorPlacement.EquallySpacedRectSide\",\"uuid\":\"701fdbad-c928-45f3-8ba2-a14f680316f8\"},{\"content\":{\"side\":\"TOP\"},\"type\":\"ConnectorPlacement.EquallySpacedRectSide\",\"uuid\":\"d648951b-caea-4569-a411-8455254fdbc0\"},{\"content\":{\"connectorIds\":[\"In2\"],\"side\":\"BOTTOM\"},\"type\":\"ConnectorPlacement.EquallySpacedRectSide\",\"uuid\":\"07eb9aa1-f407-41f0-8942-d6ed405114b5\"}]},\"type\":\"ConnectorPlacement.EquallySpacedConnector\",\"uuid\":\"7c33ff72-602e-419f-9c2d-5eefc0d60400\"}],\"packageUris\":[\"http://schema.mathworks.com/mf0/Connector/R2020b\"],\"version\":\"1.0\"}"
  M2_Comm : Subsystem
      settings: PortSchema="{\"entries\":[{\"content\":{\"sides\":[{\"content\":{\"connectorIds\":[\"In1\",\"Out2\"]},\"type\":\"ConnectorPlacement.EquallySpacedRectSide\",\"uuid\":\"47077a1e-eba1-4129-8203-93262b2de465\"},{\"content\":{\"connectorIds\":[\"Out1\",\"In3\"],\"side\":\"RIGHT\"},\"type\":\"ConnectorPlacement.EquallySpacedRectSide\",\"uuid\":\"701fdbad-c928-45f3-8ba2-a14f680316f8\"},{\"content\":{\"side\":\"TOP\"},\"type\":\"ConnectorPlacement.EquallySpacedRectSide\",\"uuid\":\"d648951b-caea-4569-a411-8455254fdbc0\"},{\"content\":{\"connectorIds\":[\"In2\"],\"side\":\"BOTTOM\"},\"type\":\"ConnectorPlacement.EquallySpacedRectSide\",\"uuid\":\"01601a56-4c3c-4c18-be21-822f443ca232\"}]},\"type\":\"ConnectorPlacement.EquallySpacedConnector\",\"uuid\":\"7c33ff72-602e-419f-9c2d-5eefc0d60400\"}],\"packageUris\":[\"http://schema.mathworks.com/mf0/Connector/R2020b\"],\"version\":\"1.0\"}"
  M3_Comm : Subsystem
      settings: PortSchema="{\"entries\":[{\"content\":{\"sides\":[{\"content\":{\"connectorIds\":[\"In1\",\"Out2\"]},\"type\":\"ConnectorPlacement.EquallySpacedRectSide\",\"uuid\":\"47077a1e-eba1-4129-8203-93262b2de465\"},{\"content\":{\"connectorIds\":[\"Out1\",\"In3\"],\"side\":\"RIGHT\"},\"type\":\"ConnectorPlacement.EquallySpacedRectSide\",\"uuid\":\"701fdbad-c928-45f3-8ba2-a14f680316f8\"},{\"content\":{\"side\":\"TOP\"},\"type\":\"ConnectorPlacement.EquallySpacedRectSide\",\"uuid\":\"d648951b-caea-4569-a411-8455254fdbc0\"},{\"content\":{\"connectorIds\":[\"In2\"],\"side\":\"BOTTOM\"},\"type\":\"ConnectorPlacement.EquallySpacedRectSide\",\"uuid\":\"b7518228-bb66-4696-b5d4-126a1140e1c3\"}]},\"type\":\"ConnectorPlacement.EquallySpacedConnector\",\"uuid\":\"7c33ff72-602e-419f-9c2d-5eefc0d60400\"}],\"packageUris\":[\"http://schema.mathworks.com/mf0/Connector/R2020b\"],\"version\":\"1.0\"}"
  M4_Comm : Subsystem
      settings: PortSchema="{\"entries\":[{\"content\":{\"sides\":[{\"content\":{\"connectorIds\":[\"In1\",\"Out2\"]},\"type\":\"ConnectorPlacement.EquallySpacedRectSide\",\"uuid\":\"47077a1e-eba1-4129-8203-93262b2de465\"},{\"content\":{\"connectorIds\":[\"Out1\",\"In3\"],\"side\":\"RIGHT\"},\"type\":\"ConnectorPlacement.EquallySpacedRectSide\",\"uuid\":\"701fdbad-c928-45f3-8ba2-a14f680316f8\"},{\"content\":{\"side\":\"TOP\"},\"type\":\"ConnectorPlacement.EquallySpacedRectSide\",\"uuid\":\"d648951b-caea-4569-a411-8455254fdbc0\"},{\"content\":{\"connectorIds\":[\"In2\"],\"side\":\"BOTTOM\"},\"type\":\"ConnectorPlacement.EquallySpacedRectSide\",\"uuid\":\"5f4b38d1-ea61-4297-b8b6-4cb7ffcc6410\"}]},\"type\":\"ConnectorPlacement.EquallySpacedConnector\",\"uuid\":\"7c33ff72-602e-419f-9c2d-5eefc0d60400\"}],\"packageUris\":[\"http://schema.mathworks.com/mf0/Connector/R2020b\"],\"version\":\"1.0\"}"
  M5_Comm : Subsystem
      settings: PortSchema="{\"entries\":[{\"content\":{\"sides\":[{\"content\":{\"connectorIds\":[\"In1\",\"Out2\"]},\"type\":\"ConnectorPlacement.EquallySpacedRectSide\",\"uuid\":\"47077a1e-eba1-4129-8203-93262b2de465\"},{\"content\":{\"connectorIds\":[\"Out1\",\"In3\"],\"side\":\"RIGHT\"},\"type\":\"ConnectorPlacement.EquallySpacedRectSide\",\"uuid\":\"701fdbad-c928-45f3-8ba2-a14f680316f8\"},{\"content\":{\"side\":\"TOP\"},\"type\":\"ConnectorPlacement.EquallySpacedRectSide\",\"uuid\":\"d648951b-caea-4569-a411-8455254fdbc0\"},{\"content\":{\"connectorIds\":[\"In2\"],\"side\":\"BOTTOM\"},\"type\":\"ConnectorPlacement.EquallySpacedRectSide\",\"uuid\":\"cd08f752-2006-4da0-88d6-bb4b20ac3ab7\"}]},\"type\":\"ConnectorPlacement.EquallySpacedConnector\",\"uuid\":\"7c33ff72-602e-419f-9c2d-5eefc0d60400\"}],\"packageUris\":[\"http://schema.mathworks.com/mf0/Connector/R2020b\"],\"version\":\"1.0\"}"
  M6_TX_signal : Outport
  M7_TX_signal : Outport  Port=2
  M8_TX_signal : Outport  Port=3
  M9_TX_signal : Outport  Port=4
  M10_TX_signal : Outport  Port=5
  wires:
  [lower_arm_info] -> M5_Comm/1(TX_variables)
  M4_Comm/1(TX_signal) -> M9_TX_signal/1
  [lower_arm_info] -> M1_Comm/1(TX_variables)
  [lower_arm_info] -> M4_Comm/1(TX_variables)
  M3_Comm/1(TX_signal) -> M8_TX_signal/1
  M2_Comm/1(TX_signal) -> M7_TX_signal/1
  [lower_arm_info] -> M2_Comm/1(TX_variables)
  [lower_arm_info] -> M3_Comm/1(TX_variables)
  M6_RX_signal/1 -> M1_Comm/3(RX_signal)
  [sync] -> M3_Comm/2(sync)
  M8_RX_signal/1 -> M3_Comm/3(RX_signal)
  [sync] -> M5_Comm/2(sync)
  [sync] -> M4_Comm/2(sync)
  [sync] -> M1_Comm/2(sync)
  M10_RX_signal/1 -> M5_Comm/3(RX_signal)
  M1_Comm/1(TX_signal) -> M6_TX_signal/1
  M7_RX_signal/1 -> M2_Comm/3(RX_signal)
  [sync] -> M2_Comm/2(sync)
  M5_Comm/1(TX_signal) -> M10_TX_signal/1
  M9_RX_signal/1 -> M4_Comm/3(RX_signal)
  lower_arm_info/1 -> [lower_arm_info]
  sync/1 -> [sync]

== system MMC_phase_centralized_HAAS_20260927/ /Communication_subsystem/Upper_arm ==
  upper_arm_info : Inport
  sync : Inport  Port=2
  M1_RX_signal : Inport  Port=3
  M2_RX_signal : Inport  Port=4
  M3_RX_signal : Inport  Port=5
  M4_RX_signal : Inport  Port=6
  M5_RX_signal : Inport  Port=7
  M1_Comm : Subsystem
      settings: PortSchema="{\"entries\":[{\"content\":{\"sides\":[{\"content\":{\"connectorIds\":[\"In1\",\"Out2\"]},\"type\":\"ConnectorPlacement.EquallySpacedRectSide\",\"uuid\":\"c3733cfa-9814-4ae5-a55a-8e5b6f8a57d7\"},{\"content\":{\"connectorIds\":[\"Out1\",\"In3\"],\"side\":\"RIGHT\"},\"type\":\"ConnectorPlacement.EquallySpacedRectSide\",\"uuid\":\"d16535d3-81ee-4162-a646-15cef1f1639a\"},{\"content\":{\"side\":\"TOP\"},\"type\":\"ConnectorPlacement.EquallySpacedRectSide\",\"uuid\":\"672d53ef-99b6-4fa6-8351-42251f607454\"},{\"content\":{\"connectorIds\":[\"In2\"],\"side\":\"BOTTOM\"},\"type\":\"ConnectorPlacement.EquallySpacedRectSide\",\"uuid\":\"a9bd7512-44c2-4af9-8132-4c17be33b3c2\"}]},\"type\":\"ConnectorPlacement.EquallySpacedConnector\",\"uuid\":\"554aea8b-7fd0-4035-ac75-3acab423d605\"}],\"packageUris\":[\"http://schema.mathworks.com/mf0/Connector/R2020b\"],\"version\":\"1.0\"}"
  M2_Comm : Subsystem
      settings: PortSchema="{\"entries\":[{\"content\":{\"sides\":[{\"content\":{\"connectorIds\":[\"In1\",\"Out2\"]},\"type\":\"ConnectorPlacement.EquallySpacedRectSide\",\"uuid\":\"47077a1e-eba1-4129-8203-93262b2de465\"},{\"content\":{\"connectorIds\":[\"Out1\",\"In3\"],\"side\":\"RIGHT\"},\"type\":\"ConnectorPlacement.EquallySpacedRectSide\",\"uuid\":\"701fdbad-c928-45f3-8ba2-a14f680316f8\"},{\"content\":{\"side\":\"TOP\"},\"type\":\"ConnectorPlacement.EquallySpacedRectSide\",\"uuid\":\"d648951b-caea-4569-a411-8455254fdbc0\"},{\"content\":{\"connectorIds\":[\"In2\"],\"side\":\"BOTTOM\"},\"type\":\"ConnectorPlacement.EquallySpacedRectSide\",\"uuid\":\"d4b1d2d6-b4a1-4e2c-9ca6-248db102ef7c\"}]},\"type\":\"ConnectorPlacement.EquallySpacedConnector\",\"uuid\":\"7c33ff72-602e-419f-9c2d-5eefc0d60400\"}],\"packageUris\":[\"http://schema.mathworks.com/mf0/Connector/R2020b\"],\"version\":\"1.0\"}"
  M3_Comm : Subsystem
      settings: PortSchema="{\"entries\":[{\"content\":{\"sides\":[{\"content\":{\"connectorIds\":[\"In1\",\"Out2\"]},\"type\":\"ConnectorPlacement.EquallySpacedRectSide\",\"uuid\":\"47077a1e-eba1-4129-8203-93262b2de465\"},{\"content\":{\"connectorIds\":[\"Out1\",\"In3\"],\"side\":\"RIGHT\"},\"type\":\"ConnectorPlacement.EquallySpacedRectSide\",\"uuid\":\"701fdbad-c928-45f3-8ba2-a14f680316f8\"},{\"content\":{\"side\":\"TOP\"},\"type\":\"ConnectorPlacement.EquallySpacedRectSide\",\"uuid\":\"d648951b-caea-4569-a411-8455254fdbc0\"},{\"content\":{\"connectorIds\":[\"In2\"],\"side\":\"BOTTOM\"},\"type\":\"ConnectorPlacement.EquallySpacedRectSide\",\"uuid\":\"e45915a7-b7a2-4a5e-b9ff-be90cdaaaa95\"}]},\"type\":\"ConnectorPlacement.EquallySpacedConnector\",\"uuid\":\"7c33ff72-602e-419f-9c2d-5eefc0d60400\"}],\"packageUris\":[\"http://schema.mathworks.com/mf0/Connector/R2020b\"],\"version\":\"1.0\"}"
  M4_Comm : Subsystem
      settings: PortSchema="{\"entries\":[{\"content\":{\"sides\":[{\"content\":{\"connectorIds\":[\"In1\",\"Out2\"]},\"type\":\"ConnectorPlacement.EquallySpacedRectSide\",\"uuid\":\"47077a1e-eba1-4129-8203-93262b2de465\"},{\"content\":{\"connectorIds\":[\"Out1\",\"In3\"],\"side\":\"RIGHT\"},\"type\":\"ConnectorPlacement.EquallySpacedRectSide\",\"uuid\":\"701fdbad-c928-45f3-8ba2-a14f680316f8\"},{\"content\":{\"side\":\"TOP\"},\"type\":\"ConnectorPlacement.EquallySpacedRectSide\",\"uuid\":\"d648951b-caea-4569-a411-8455254fdbc0\"},{\"content\":{\"connectorIds\":[\"In2\"],\"side\":\"BOTTOM\"},\"type\":\"ConnectorPlacement.EquallySpacedRectSide\",\"uuid\":\"fe4854bf-7531-4052-9f9a-05b48e3d1945\"}]},\"type\":\"ConnectorPlacement.EquallySpacedConnector\",\"uuid\":\"7c33ff72-602e-419f-9c2d-5eefc0d60400\"}],\"packageUris\":[\"http://schema.mathworks.com/mf0/Connector/R2020b\"],\"version\":\"1.0\"}"
  M5_Comm : Subsystem
      settings: PortSchema="{\"entries\":[{\"content\":{\"sides\":[{\"content\":{\"connectorIds\":[\"In1\",\"Out2\"]},\"type\":\"ConnectorPlacement.EquallySpacedRectSide\",\"uuid\":\"47077a1e-eba1-4129-8203-93262b2de465\"},{\"content\":{\"connectorIds\":[\"Out1\",\"In3\"],\"side\":\"RIGHT\"},\"type\":\"ConnectorPlacement.EquallySpacedRectSide\",\"uuid\":\"701fdbad-c928-45f3-8ba2-a14f680316f8\"},{\"content\":{\"side\":\"TOP\"},\"type\":\"ConnectorPlacement.EquallySpacedRectSide\",\"uuid\":\"d648951b-caea-4569-a411-8455254fdbc0\"},{\"content\":{\"connectorIds\":[\"In2\"],\"side\":\"BOTTOM\"},\"type\":\"ConnectorPlacement.EquallySpacedRectSide\",\"uuid\":\"76d1056e-e7b2-4023-89b8-57825a028de1\"}]},\"type\":\"ConnectorPlacement.EquallySpacedConnector\",\"uuid\":\"7c33ff72-602e-419f-9c2d-5eefc0d60400\"}],\"packageUris\":[\"http://schema.mathworks.com/mf0/Connector/R2020b\"],\"version\":\"1.0\"}"
  M1_TX_signal : Outport
  M2_TX_signal : Outport  Port=2
  M3_TX_signal : Outport  Port=3
  M4_TX_signal : Outport  Port=4
  M5_TX_signal : Outport  Port=5
  RX_Variables : Outport  Port=6
  wires:
  [upper_arm_info] -> M5_Comm/1(TX_variables)
  M4_Comm/1(TX_signal) -> M4_TX_signal/1
  [upper_arm_info] -> M1_Comm/1(TX_variables)
  [upper_arm_info] -> M4_Comm/1(TX_variables)
  M3_Comm/1(TX_signal) -> M3_TX_signal/1
  M2_Comm/1(TX_signal) -> M2_TX_signal/1
  [upper_arm_info] -> M2_Comm/1(TX_variables)
  [upper_arm_info] -> M3_Comm/1(TX_variables)
  M1_RX_signal/1 -> M1_Comm/3(RX_signal)
  [sync] -> M3_Comm/2(sync)
  M3_RX_signal/1 -> M3_Comm/3(RX_signal)
  [sync] -> M5_Comm/2(sync)
  [sync] -> M4_Comm/2(sync)
  [sync] -> M1_Comm/2(sync)
  M5_RX_signal/1 -> M5_Comm/3(RX_signal)
  M1_Comm/1(TX_signal) -> M1_TX_signal/1
  M2_RX_signal/1 -> M2_Comm/3(RX_signal)
  [sync] -> M2_Comm/2(sync)
  M5_Comm/1(TX_signal) -> M5_TX_signal/1
  M4_RX_signal/1 -> M4_Comm/3(RX_signal)
  upper_arm_info/1 -> [upper_arm_info]
  sync/1 -> [sync]
  M1_Comm/2(RX_Variables) -> RX_Variables/1

== system MMC_phase_centralized_HAAS_20260927/ /Sinus Modulation + Sorting Algorithm/M1 MCU ==
  g_u : Inport
  M_number : Inport  Port=2
  CVB_upper : MATLAB Function  TreatAsAtomicUnit=on
  g_unitaire_stack : Outport
  wires:
  g_u/1 -> CVB_upper/1(g)
  M_number/1 -> CVB_upper/2(M_number)
  CVB_upper/1(y) -> g_unitaire_stack/1

== system MMC_phase_centralized_HAAS_20260927/ /Sinus Modulation + Sorting Algorithm/M2 MCU ==
  g_u : Inport
  M_number : Inport  Port=2
  CVB_upper : MATLAB Function  TreatAsAtomicUnit=on
  g_unitaire_stack : Outport
  wires:
  g_u/1 -> CVB_upper/1(g)
  M_number/1 -> CVB_upper/2(M_number)
  CVB_upper/1(y) -> g_unitaire_stack/1

== system MMC_phase_centralized_HAAS_20260927/ /Sinus Modulation + Sorting Algorithm/M3 MCU ==
  g_u : Inport
  M_number : Inport  Port=2
  CVB_upper : MATLAB Function  TreatAsAtomicUnit=on
  g_unitaire_stack : Outport
  wires:
  g_u/1 -> CVB_upper/1(g)
  M_number/1 -> CVB_upper/2(M_number)
  CVB_upper/1(y) -> g_unitaire_stack/1

== system MMC_phase_centralized_HAAS_20260927/ /Sinus Modulation + Sorting Algorithm/M4 MCU ==
  g_u : Inport
  M_number : Inport  Port=2
  CVB_upper : MATLAB Function  TreatAsAtomicUnit=on
  g_unitaire_stack : Outport
  wires:
  g_u/1 -> CVB_upper/1(g)
  M_number/1 -> CVB_upper/2(M_number)
  CVB_upper/1(y) -> g_unitaire_stack/1

== system MMC_phase_centralized_HAAS_20260927/ /Sinus Modulation + Sorting Algorithm/M5 MCU ==
  g_u : Inport
  M_number : Inport  Port=2
  CVB_upper : MATLAB Function  TreatAsAtomicUnit=on
  g_unitaire_stack : Outport
  wires:
  g_u/1 -> CVB_upper/1(g)
  M_number/1 -> CVB_upper/2(M_number)
  CVB_upper/1(y) -> g_unitaire_stack/1
